simulink model "Comprobacion_Final"  (R2024a)
settings: Solver=ode45  StartTime=0.0  StopTime=10  MaxStep=0.001  RelTol=1e-3
(part 1 of 2)
settings Model: Creator=Usuario  LastModifiedBy=Usuario
settings ModelReferenceCC: UpdateModelReferenceTargets=IfOutOfDate
settings RTWCC: GPUComputeCapability=7.5
settings ConfigComp: CovMetricSettings=de  CovBoundaryAbsTol=1.0e-5

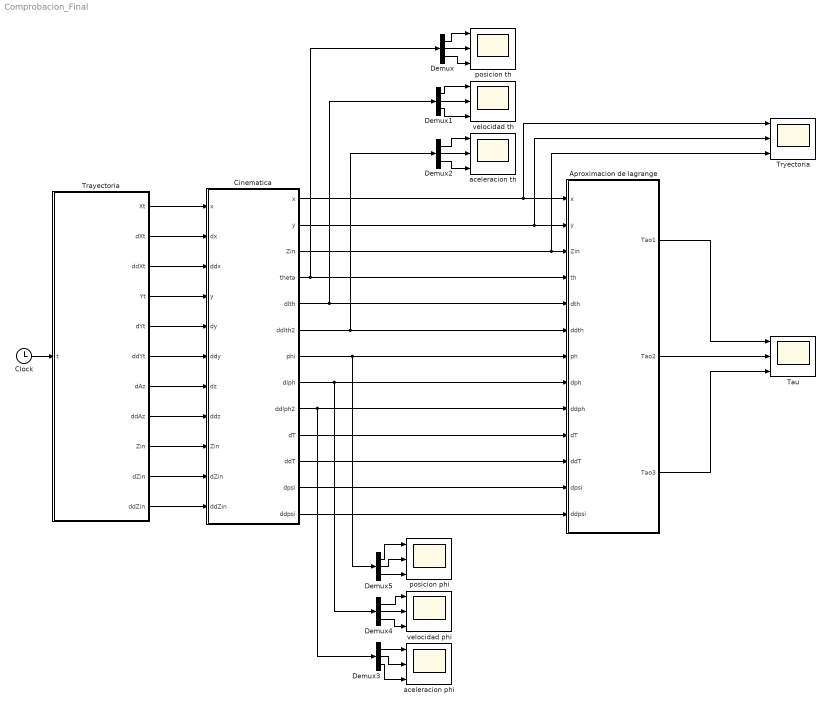
== system Comprobacion_Final ==
  Aproximacion de lagrange : MATLAB Function  TreatAsAtomicUnit=on
  Cinematica : MATLAB Function  TreatAsAtomicUnit=on
  Clock : Clock
  Demux{,1..5} (6 alike) : Demux  Outputs=3
  Tau : Scope  NumInputPorts=3
  Trayectoria : MATLAB Function  TreatAsAtomicUnit=on
  Tryectoria : Scope  NumInputPorts=3
  aceleracion phi : Scope  NumInputPorts=3
  aceleracion th : Scope  NumInputPorts=3
  posicion phi : Scope  NumInputPorts=3
  posicion th : Scope  NumInputPorts=3
  velocidad phi : Scope  NumInputPorts=3
  velocidad th : Scope  NumInputPorts=3
  wires:
  Demux5/3 -> posicion phi/3
  Demux5/2 -> posicion phi/2
  Demux4/3 -> velocidad phi/3
  Demux5/1 -> posicion phi/1
  Demux4/1 -> velocidad phi/1
  Aproximacion de lagrange/2(Tao2) -> Tau/2
  Aproximacion de lagrange/3(Tao3) -> Tau/3
  Aproximacion de lagrange/1(Tao1) -> Tau/1
  Demux3/2 -> aceleracion phi/2
  Demux3/3 -> aceleracion phi/3
  Demux3/1 -> aceleracion phi/1
  Demux2/1 -> aceleracion th/1
  Demux/2 -> posicion th/2
  Demux/1 -> posicion th/1
  Demux1/1 -> velocidad th/1
  Demux2/3 -> aceleracion th/3
  Cinematica/1(x) -> Tryectoria/1, Aproximacion de lagrange/1(x)
  Cinematica/2(y) -> Tryectoria/2, Aproximacion de lagrange/2(y)
  Cinematica/3(Zin) -> Tryectoria/3, Aproximacion de lagrange/3(Zin)
  Cinematica/8(dlph) -> Demux4/1, Aproximacion de lagrange/8(dph)
  Demux4/2 -> velocidad phi/2
  Demux1/3 -> velocidad th/3
  Demux1/2 -> velocidad th/2
  Demux2/2 -> aceleracion th/2
  Demux/3 -> posicion th/3
  Cinematica/5(dlth) -> Demux1/1, Aproximacion de lagrange/5(dth)
  Clock/1 -> Trayectoria/1(t)
  Cinematica/4(theta) -> Demux/1, Aproximacion de lagrange/4(th)
  Cinematica/7(phi) -> Demux5/1, Aproximacion de lagrange/7(ph)
  Cinematica/6(ddlth2) -> Demux2/1, Aproximacion de lagrange/6(ddth)
  Cinematica/9(ddlph2) -> Demux3/1, Aproximacion de lagrange/9(ddph)
  Cinematica/10(dT) -> Aproximacion de lagrange/10(dT)
  Cinematica/11(ddT) -> Aproximacion de lagrange/11(ddT)
  Cinematica/12(dpsi) -> Aproximacion de lagrange/12(dpsi)
  Cinematica/13(ddpsi) -> Aproximacion de lagrange/13(ddpsi)
  Trayectoria/1(Xt) -> Cinematica/1("x ")
  Trayectoria/2(dXt) -> Cinematica/2(dx)
  Trayectoria/3(ddXt) -> Cinematica/3(ddx)
  Trayectoria/4(Yt) -> Cinematica/4("y ")
  Trayectoria/5(dYt) -> Cinematica/5(dy)
  Trayectoria/6(ddYt) -> Cinematica/6(ddy)
  Trayectoria/7(dAz) -> Cinematica/7(dz)
  Trayectoria/8(ddAz) -> Cinematica/8(ddz)
  Trayectoria/9(Zin) -> Cinematica/9("Zin ")
  Trayectoria/10(dZin) -> Cinematica/10(dZin)
  Trayectoria/11(ddZin) -> Cinematica/11(ddZin)

== matlab function Comprobacion_Final/Aproximacion de lagrange ==
  data: Tao1 output size=[1,1]; Tao2 output size=[1,1]; Tao3 output size=[1,1]; x input size=[1,1]; y input size=[1,1]; Zin input size=[1,1]; th input size=[3,1]; dth input size=[3,1]; ddth input size=[3,1]; ph input size=[3,1]; dph input size=[3,1]; ddph input size=[3,1]; dT input size=[3,1]; ddT input size=[3,1]; dpsi input size=[3,1]; ddpsi input size=[3,1]
function [Tao1, Tao2, Tao3] = fcn(x, y, Zin, th, dth, ddth, ph, dph, ddph, dT,ddT,dpsi, ddpsi)
%%constantes
p  = 55; %mm   
b  = 50;    
l1 = 45;   
l2 = 75;  
d1 = 19.718; 
d2 = 36.703;
dp = 52.00;
m1 = 3.18; %gramos
m2 = 4.36;
mp = 43.32;
I1yy = 652.49;
I2yy = 519.69;
IPx = 21311.68;
IPy = 42281.84;
IPz = 21311.66;
g = 9810; %mm/s2
%% ============================================================
Ax = x;
Ay = y;
f1=(-sin(Ax)*sin(Ay))/(cos(Ax)+cos(Ay));
Az=atan(f1);

alfa1 = deg2rad(0);
alfa2 = deg2rad(120);
alfa3 = deg2rad(240);
R = [ cos(Ay)*cos(Az)                          -cos(Ay)*sin(Az)                          sin(Ay)
    cos(Ax)*sin(Az)+cos(Az)*sin(Ax)*sin(Ay)    cos(Ax)*cos(Az)-sin(Ax)*sin(Ay)*sin(Az)  -cos(Ay)*sin(Ax)
    sin(Ax)*sin(Az)-cos(Ax)*cos(Az)*sin(Ay)    cos(Az)*sin(Ax)+cos(Ax)*sin(Ay)*sin(Az)   cos(Ax)*cos(Ay)];
ux = R(1,1); uy = R(1,2); vy = R(2,2);
Ox = (p*(ux-vy))/2;
Oy = -uy*p;
Oz = Zin;
T = [Ox;Oy;Oz];
psi = [Ax; Ay; Az];
psix=Ax; psiy=Ay; psiz=Az; 

th1 = th(1); th2 = th(2); th3 = th(3);
dth1 = dth(1); dth2 = dth(2); dth3 = dth(3);
ddth1 = ddth(1); ddth2 = ddth(2); ddth3 = ddth(3);
ph1 = ph(1); ph2 = ph(2); ph3 = ph(3);
dph1 = dph(1); dph2 = dph(2); dph3 = dph(3);
ddph1 = ddph(1); ddph2 = ddph(2); ddph3 = ddph(3);
dpsix = dpsi(1); dpsiy = dpsi(2); dpsiz = dpsi(3);
ddpsix = ddpsi(1); ddpsiy = ddpsi(2); ddpsiz = ddpsi(3);
dOx = dT(1); dOy = dT(2); dOz = dT(3);
ddOx = ddT(1); ddOy = ddT(2); ddOz = ddT(3);
%% lagrangiano
L1 = g*(-d1*m1 - l2*m2)*cos(th1) + d2*l2*m2*sin(th1 - ph1)*dph1^2+ (I1yy + d1^2*m1 + l2^2*m2)*ddth1 + d2*l2*m2*cos(th1 - ph1)*ddph1;
L2 = g*(-d1*m1 - l2*m2)*cos(th2) + d2*l2*m2*sin(th2 - ph2)*dph2^2+ (I1yy + d1^2*m1 + l2^2*m2)*ddth2 + d2*l2*m2*cos(th2 - ph2)*ddph2;
L3 = g*(-d1*m1 - l2*m2)*cos(th3) + d2*l2*m2*sin(th3 - ph3)*dph3^2+ (I1yy + d1^2*m1 + l2^2*m2)*ddth3 + d2*l2*m2*cos(th3 - ph3)*ddph3;
L4 = -d2*g*m2*cos(ph1) + I2yy*ddph1 + d2*m2*(-l2*sin(th1 - ph1)*dth1^2 + l2*cos(th1 - ph1)*ddth1 + d2*ddph1);
L5 = -d2*g*m2*cos(ph2) + I2yy*ddph2 + d2*m2*(-l2*sin(th2 - ph2)*dth2^2 + l2*cos(th2 - ph2)*ddth2 + d2*ddph2);
L6 = -d2*g*m2*cos(ph3) + I2yy*ddph3 + d2*m2*(-l2*sin(th3 - ph3)*dth3^2 + l2*cos(th3 - ph3)*ddth3 + d2*ddph3);
L7 = mp*(-dp*sin(psiy)*dpsiy^2 + ddOx + dp*cos(psiy)*ddpsiy);
L8 = mp*(ddOy + dp*(sin(psix)*cos(psiy)*dpsix^2 + 2*cos(psix)*sin(psiy)*dpsix*dpsiy + sin(psix)*cos(psiy)*dpsiy^2 - cos(psix)*cos(psiy)*ddpsix + sin(psix)*sin(psiy)*ddpsiy));
L9 = mp*(g + ddOz + dp*(- cos(psix)*cos(psiy)*dpsix^2 + 2*sin(psix)*sin(psiy)*dpsix*dpsiy + cos(psix)*cos(psiy)*dpsiy^2 - sin(psix)*cos(psiy)*ddpsix - cos(psix)*sin(psiy)*ddpsiy));
L10 = -dp*g*mp*sin(psix)*cos(psiy) - dp^2*mp*sin(2*psiy)*dpsix*dpsiy + 0.5*(IPy - IPz)*sin(2*psix)*dpsiy^2 - dp*mp*cos(psix)*cos(psiy)*ddOy + (IPx + (IPy - IPz)*cos(2*psix))*cos(psiy)*dpsiy*dpsiz - IPy*cos(psix)*sin(psix)*cos(psiy)^2*dpsiz^2 + 0.5*IPz*sin(2*psix)*cos(psiy)^2*dpsiz^2 - dp*mp*sin(psix)*cos(psiy)*ddOz + IPx*ddpsix + 0.5*dp^2*mp*ddpsix + 0.5*dp^2*mp*cos(2*psiy)*ddpsix + IPx*sin(psiy)*ddpsiz;
L11 = -dp*g*mp*cos(psix)*sin(psiy) + 0.5*dp^2*mp*sin(2*psiy)*dpsix^2 + 0.5*(IPz*cos(psix)^2*sin(2*psiy) + (-IPx + IPy*sin(psix)^2)*sin(2*psiy) )*dpsiz^2 + dpsix*(-IPx*cos(psiy)*dpsiz + (-IPy + IPz)*(sin(2*psix)*dpsiy + cos(2*psix)*cos(psiy)*dpsiz)) + dp*mp*cos(psiy)*ddOx + dp*mp*sin(psix)*sin(psiy)*ddOy - dp*mp*cos(psix)*sin(psiy)*ddOz + 0.5*(IPy + IPz)*ddpsiy + dp^2*mp*ddpsiy + 0.5*cos(2*psix)*(IPy - IPz)*ddpsiy - 0.5*sin(2*psix)*cos(psiy)*(IPy - IPz)*ddpsiz;
L12 = 0.5*(IPy - IPz)*sin(2*psix)*sin(psiy)*dpsiy^2 + (-IPz*cos(psix)^2 + (IPx - IPy*sin(psix)^2))*sin(2*psiy)*dpsiy*dpsiz + (IPx + (-IPy + IPz)*cos(2*psix))*cos(psiy)*dpsix*dpsiy + (IPy - IPz)*sin(2*psix)*cos(psiy)^2*dpsix*dpsiz + (0.5*(-IPy + IPz)*sin(2*psix)*cos(psiy)*ddpsiy + (IPz*cos(psix)^2 + IPy*sin(psix)^2)*cos(psiy)^2*ddpsiz) + IPx*sin(psiy)*(ddpsix + sin(psiy)*ddpsiz);

Lagrange1=[L1;L2;L3];
Lagrange2=[L4;L5;L6;L7;L8;L9;L10;L11;L12]; %Fuerzas externas sobre L7, L8, L9 (x,y,z)
%% matriz gamma
Gamma1 = ...
[-l1*cos(alfa1)*sin(th1), -l1*sin(alfa1)*sin(th1), l1*cos(th1),                                                                                 0,                                                                                 0,                                             0,                                                                                 0,                                                                                 0,                                               0
                       0,                       0,           0,                                                           -l1*cos(alfa2)*sin(th2),                                                           -l1*sin(alfa2)*sin(th2),                                   l1*cos(th2),                                                                                 0,                                                                                 0,                                               0
                       0,                       0,           0,                                                                                 0,                                                                                 0,                                             0,                                                           -l1*cos(alfa3)*sin(th3),                                                           -l1*sin(alfa3)*sin(th3),                                     l1*cos(th3)];
Gamma2 = ...
[-l2*cos(alfa1)*sin(ph1), -l2*sin(alfa1)*sin(ph1), l2*cos(ph1),                                                                                 0,                                                                                 0,                                             0,                                                                                 0,                                                                                 0,                                               0
                       0,                       0,           0,                                                           -l2*cos(alfa2)*sin(ph2),                                                           -l2*sin(alfa2)*sin(ph2),                                   l2*cos(ph2),                                                                                 0,                                                                                 0,                                               0
                       0,                       0,           0,                                                                                 0,                                                                                 0,                                             0,                                                           -l2*cos(alfa3)*sin(ph3),                                                           -l2*sin(alfa3)*sin(ph3),                                     l2*cos(ph3)
                       1,                       0,           0,                                                                                 1,                                                                                 0,                                             0,                                                                                 1,                                                                                 0,                                               0
                       0,                       1,           0,                                                                                 0,                                                                                 1,                                             0,                                                                                 0,                                                                                 1,                                               0
                       0,                       0,           1,                                                                                 0,                                                                                 0,                                             1,                                                                                 0,                                                                                 0,                                               1
                       0,                       0,           0,                        -(3^(1/2)*p*(sin(Ax)*sin(Az) - cos(Ax)*cos(Az)*sin(Ay)))/2,                        -(3^(1/2)*p*(cos(Az)*sin(Ax) + cos(Ax)*sin(Ay)*sin(Az)))/2,                -(3^(1/2)*p*cos(Ax)*cos(Ay))/2,                         (3^(1/2)*p*(sin(Ax)*sin(Az) - cos(Ax)*cos(Az)*sin(Ay)))/2,                         (3^(1/2)*p*(cos(Az)*sin(Ax) + cos(Ax)*sin(Ay)*sin(Az)))/2,                   (3^(1/2)*p*cos(Ax)*cos(Ay))/2
      -p*cos(Az)*sin(Ay),       p*sin(Ay)*sin(Az),   p*cos(Ay),                     (p*cos(Az)*sin(Ay))/2 + (3^(1/2)*p*cos(Ay)*cos(Az)*sin(Ax))/2,                   - (p*sin(Ay)*sin(Az))/2 - (3^(1/2)*p*cos(Ay)*sin(Ax)*sin(Az))/2, (3^(1/2)*p*sin(Ax)*sin(Ay))/2 - (p*cos(Ay))/2,                     (p*cos(Az)*sin(Ay))/2 - (3^(1/2)*p*cos(Ay)*cos(Az)*sin(Ax))/2,                     (3^(1/2)*p*cos(Ay)*sin(Ax)*sin(Az))/2 - (p*sin(Ay)*sin(Az))/2, - (p*cos(Ay))/2 - (3^(1/2)*p*sin(Ax)*sin(Ay))/2
      -p*cos(Ay)*sin(Az),      -p*cos(Ay)*cos(Az),           0, (p*cos(Ay)*sin(Az))/2 + (3^(1/2)*p*(cos(Ax)*cos(Az) - sin(Ax)*sin(Ay)*sin(Az)))/2, (p*cos(Ay)*cos(Az))/2 - (3^(1/2)*p*(cos(Ax)*sin(Az) + cos(Az)*sin(Ax)*sin(Ay)))/2,                                             0, (p*cos(Ay)*sin(Az))/2 - (3^(1/2)*p*(cos(Ax)*cos(Az) - sin(Ax)*sin(Ay)*sin(Az)))/2, (p*cos(Ay)*cos(Az))/2 + (3^(1/2)*p*(cos(Ax)*sin(Az) + cos(Az)*sin(Ax)*sin(Ay)))/2,                                               0];

%% Matriz lambda y torques
Lambda= (inv(Gamma2))*Lagrange2;
Ta= Lagrange1 + Gamma1*Lambda;
Tao= Ta*10^-9;
Tao1=Tao(1); Tao2=Tao(2); Tao3=Tao(3);
end

== matlab function Comprobacion_Final/Trayectoria ==
  data: Xt output; dXt output; ddXt output; Yt output; dYt output; ddYt output; dAz output; ddAz output; Zin output; t input; dZin output; ddZin output
function [Xt,dXt,ddXt, Yt,dYt,ddYt, dAz, ddAz, Zin,dZin,ddZin] = fcn(t)
%% Trayectoria
w   = 0.25*pi;       % frecuencia angular [rad/s]
amp = deg2rad(10);  % amplitud ±10 grados convertida a radianes

t1 = 5;        % fin rampa de subida (60 -> 75)
t2 = 15;       % fin de la fase senoidal (10 s)
t3 = 20;       % fin rampa de bajada (75 -> 60)

if t < t1
    % Rampa de subida: Z va de 60 a 75 en 5 s
    Zin   = 60 + 47.95*(t/t1);
    dZin  = 15/t1;
    ddZin = 0;

    Xt = 0;  Yt = 0;
    dXt = 0; dYt = 0;
    ddXt = 0; ddYt = 0;
    R = (cos(Xt) + cos(Yt))^2 + sin(Xt)^2*sin(Yt)^2;
    Q = -dXt*sin(Yt)*cos(Yt)-dYt*sin(Xt)*cos(Xt);
    dAz = Q/R;
    dQ = -ddXt*sin(Yt)*cos(Yt)-dXt*dYt*cos(2*Yt)-ddYt*sin(Xt)*cos(Xt)-dYt*dXt*cos(2*Xt);
    dR = 2*(cos(Xt)+cos(Yt))*(-sin(Xt)*dXt - sin(Yt)*dYt)+ 2*sin(Xt)*cos(Xt)*dXt*sin(Yt)^2+ 2*sin(Yt)*cos(Yt)*dYt*sin(Xt)^2;
    ddAz = (dQ*R - Q*dR)/R^2;
elseif t < t2
    % Z estable en 75, X,Y en seno puro (sin envolvente)
    Zin   = 107.95;
    dZin  = 0;
    ddZin = 0;

    tau = t - t1;

    Xt = amp*cos(w*tau);
    Yt = amp*sin(w*tau);

    dXt = -amp*w*sin(w*tau);
    dYt =  amp*w*cos(w*tau);

    ddXt = -amp*w^2*cos(w*tau);
    ddYt = -amp*w^2*sin(w*tau);

    R = (cos(Xt) + cos(Yt))^2 + sin(Xt)^2*sin(Yt)^2;
    Q = -dXt*sin(Yt)*cos(Yt)-dYt*sin(Xt)*cos(Xt);
    dAz = Q/R;
    dQ = -ddXt*sin(Yt)*cos(Yt)-dXt*Yt*cos(2*Yt)-ddYt*sin(Xt)*cos(Xt)-dYt*dXt*cos(2*Xt);
    dR = 2*(cos(Xt)+cos(Yt))*(-sin(Xt)*dXt - sin(Yt)*dYt)+ 2*sin(Xt)*cos(Xt)*dXt*sin(Yt)^2+ 2*sin(Yt)*cos(Yt)*dYt*sin(Xt)^2;
    ddAz = (dQ*R - Q*dR)/R^2;
elseif t < t3
    % Rampa de bajada: Z vuelve de 75 a 60 en 5 s, X,Y ya en 0
    Zin   = 107.95 - 47.95*((t - t2)/(t3 - t2));
    dZin  = -15/(t3 - t2);
    ddZin = 0;

    Xt = 0;  Yt = 0;
    dXt = 0; dYt = 0;
    ddXt = 0; ddYt = 0;

    R = (cos(Xt) + cos(Yt))^2 + sin(Xt)^2*sin(Yt)^2;
    Q = -dXt*sin(Yt)*cos(Yt)-dYt*sin(Xt)*cos(Xt);
    dAz = Q/R;
    dQ = -ddXt*sin(Yt)*cos(Yt)-dXt*dYt*cos(2*Yt)-ddYt*sin(Xt)*cos(Xt)-dYt*dXt*cos(2*Xt);
    dR = 2*(cos(Xt)+cos(Yt))*(-sin(Xt)*dXt - sin(Yt)*dYt)+ 2*sin(Xt)*cos(Xt)*dXt*sin(Yt)^2+ 2*sin(Yt)*cos(Yt)*dYt*sin(Xt)^2;
    ddAz = (dQ*R - Q*dR)/R^2;
else
    % Reposo final en el punto inicial
    Zin = 60; dZin = 0; ddZin = 0;
    Xt = 0;  Yt = 0;
    dXt = 0; dYt = 0;
    ddXt = 0; ddYt = 0; 
    R = (cos(Xt) + cos(Yt))^2 + sin(Xt)^2*sin(Yt)^2;
    Q = -dXt*sin(Yt)*cos(Yt)-dYt*sin(Xt)*cos(Xt);
    dAz = Q/R;
    dQ = -ddXt*sin(Yt)*cos(Yt)-dXt*dYt*cos(2*Yt)-ddYt*sin(Xt)*cos(Xt)-dYt*dXt*cos(2*Xt);
    dR = 2*(cos(Xt)+cos(Yt))*(-sin(Xt)*dXt - sin(Yt)*dYt)+ 2*sin(Xt)*cos(Xt)*dXt*sin(Yt)^2+ 2*sin(Yt)*cos(Yt)*dYt*sin(Xt)^2;
    ddAz = (dQ*R - Q*dR)/R^2;
end

end
